simulink model "Template_v5_0_0_2026a_Original"  (R2026a)
settings: Solver=ode4  StopTime=tsim  FixedStep=baseRate  RelTol=1e-6  AbsTol=1e-6
undefined symbols (not defined in the file or in its folder): baseRate, dataRate, DiscIntNeverNeededParam, F_thrusters_BLACK, F_thrusters_BLUE, F_thrusters_RED, home_states_BLACK, home_states_BLUE, home_states_RED, IBLACK, IBLUE, init_states_BLACK, init_states_BLUE, init_states_RED, IRED, K_BLACK, K_BLUE, K_RED, labConsoleIP, mBLACK, mBLUE, mRED, Phase0_End, Phase1_End, Phase2_End, Phase3_End, Phase3_SubPhase1_End, Phase3_SubPhase2_End, Phase3_SubPhase3_End, Phase3_SubPhase4_End, Phase4_End, Phase5_End, platformSelection, PWMFreq, serverRate, simMode, tableDamping_BLACK, tableDamping_BLUE, tableDamping_RED, tableSlope, thrust_decay_BLACK, thrust_decay_BLUE, thrust_decay_RED, thruster_dist2CG_BLACK, thruster_dist2CG_BLUE, thruster_dist2CG_RED, xLength, yLength
libraries: simulink x18, dspinverses x3, nvidiaCommlib x1
(part 6 of 7)

== system Template_v5_0_0_2026a_Original/Simulate Plant Dynamics/RED and ARM Dynamics/RED + ARM/Calculated & Store Measured States/Subsystem3 ==
  dt : Inport
  y : Inport  Port=2
  Constant3 : Constant  Value=0
  Delay1 : Delay  DelayLength=1
  Enabled Subsystem : Subsystem  TreatAsAtomicUnit=on
  Relational Operator : RelationalOperator  Operator=~=  OutDataTypeStr=boolean  RndMeth=Simplest  InputSameDT=off
  Subtract1 : Sum  Inputs=+-
  dy/dt : Outport
  wires:
  Constant3/1 -> Relational Operator/2
  Relational Operator/1 -> Enabled Subsystem/Enable
  Delay1/1 -> Subtract1/2
  dt/1 -> Enabled Subsystem/2(dt)
  Subtract1/1 -> Relational Operator/1
  Enabled Subsystem/1(dy/dt) -> dy/dt/1
  y/1 -> Enabled Subsystem/1(y), Delay1/1, Subtract1/1

== system Template_v5_0_0_2026a_Original/Simulate Plant Dynamics/RED and ARM Dynamics/RED + ARM/Calculated & Store Measured States/Subsystem4 ==
  dt : Inport
  y : Inport  Port=2
  Constant3 : Constant  Value=0
  Delay1 : Delay  DelayLength=1
  Enabled Subsystem : Subsystem  TreatAsAtomicUnit=on
  Relational Operator : RelationalOperator  Operator=~=  OutDataTypeStr=boolean  RndMeth=Simplest  InputSameDT=off
  Subtract1 : Sum  Inputs=+-
  dy/dt : Outport
  wires:
  Constant3/1 -> Relational Operator/2
  Relational Operator/1 -> Enabled Subsystem/Enable
  Delay1/1 -> Subtract1/2
  dt/1 -> Enabled Subsystem/2(dt)
  Subtract1/1 -> Relational Operator/1
  Enabled Subsystem/1(dy/dt) -> dy/dt/1
  y/1 -> Enabled Subsystem/1(y), Delay1/1, Subtract1/1

== system Template_v5_0_0_2026a_Original/Simulate Plant Dynamics/RED and ARM Dynamics/RED + ARM/Calculated & Store Measured States/Subsystem5 ==
  dt : Inport
  y : Inport  Port=2
  Constant3 : Constant  Value=0
  Delay1 : Delay  DelayLength=1
  Enabled Subsystem : Subsystem  TreatAsAtomicUnit=on
  Relational Operator : RelationalOperator  Operator=~=  OutDataTypeStr=boolean  RndMeth=Simplest  InputSameDT=off
  Subtract1 : Sum  Inputs=+-
  dy/dt : Outport
  wires:
  Constant3/1 -> Relational Operator/2
  Relational Operator/1 -> Enabled Subsystem/Enable
  Delay1/1 -> Subtract1/2
  dt/1 -> Enabled Subsystem/2(dt)
  Subtract1/1 -> Relational Operator/1
  Enabled Subsystem/1(dy/dt) -> dy/dt/1
  y/1 -> Enabled Subsystem/1(y), Delay1/1, Subtract1/1

== system Template_v5_0_0_2026a_Original/Simulate Plant Dynamics/RED and ARM Dynamics/RED + ARM/Calculated & Store Measured States/Wrap ==
  Unwrapped Angle : Inport
  Atan2 : Trigonometry  Operator=atan2
  Cos : Trigonometry  Operator=cos
  Sin : Trigonometry
  Wrapped Angle : Outport
  wires:
  Unwrapped Angle/1 -> Sin/1, Cos/1
  Cos/1 -> Atan2/2
  Atan2/1 -> Wrapped Angle/1
  Sin/1 -> Atan2/1

== system Template_v5_0_0_2026a_Original/Simulate Plant Dynamics/RED and ARM Dynamics/RED + ARM/Calculated & Store True States/Wrap ==
  Unwrapped Angle : Inport
  Atan2 : Trigonometry  Operator=atan2
  Cos : Trigonometry  Operator=cos
  Sin : Trigonometry
  Wrapped Angle : Outport
  wires:
  Unwrapped Angle/1 -> Sin/1, Cos/1
  Cos/1 -> Atan2/2
  Atan2/1 -> Wrapped Angle/1
  Sin/1 -> Atan2/1

== system Template_v5_0_0_2026a_Original/Simulate Plant Dynamics/RED and ARM Dynamics/RED + ARM/Data @ Measurement Rate/Calculate True Time Step ==
  Data : Inport
  Time : Inport  Port=2
  Rate : Inport  Port=3
  Constant3 : Constant  Value=0
  Delay1 : Delay  DelayLength=1  InitialCondition=0
  Delay2 : Delay  DelayLength=1  InitialCondition=0
  Demux : Demux  Outputs=[1,5]
  Enabled Subsystem3 : Subsystem  TreatAsAtomicUnit=on
  MATLAB Function : MATLAB Function  TreatAsAtomicUnit=on
  Relational Operator : RelationalOperator  Operator=~=  OutDataTypeStr=boolean  RndMeth=Simplest  InputSameDT=off
  Subtract1 : Sum  Inputs=+-
  Subtract2 : Sum  Inputs=+-
  Terminator : Terminator
  dt_out : Outport
  wires:
  Rate/1 -> MATLAB Function/2(dataRate)
  MATLAB Function/1(dt_out) -> dt_out/1
  Time/1 -> Delay2/1, Subtract1/1
  Enabled Subsystem3/1(dy(t)/dt) -> MATLAB Function/1(dt)
  Data/1 -> Demux/1
  Subtract2/1 -> Relational Operator/1
  Relational Operator/1 -> Enabled Subsystem3/Enable
  Constant3/1 -> Relational Operator/2
  Demux/1 -> Subtract2/1, Delay1/1
  Delay1/1 -> Subtract2/2
  Demux/2 -> Terminator/1
  Subtract1/1 -> Enabled Subsystem3/1(y2-y1)
  Delay2/1 -> Subtract1/2

== system Template_v5_0_0_2026a_Original/Simulate Plant Dynamics/RED and ARM Dynamics/RED + ARM/Data @ Measurement Rate/Enabled Subsystem ==
  In1 : Inport
  Enable : EnablePort
  Out1 : Outport
  wires:
  In1/1 -> Out1/1

== system Template_v5_0_0_2026a_Original/Simulate Plant Dynamics/RED and ARM Dynamics/RED + ARM/Data @ Measurement Rate/Enabled Subsystem1 ==
  ThrustPer_Final : Inport
  Enable : EnablePort
  Out1 : Outport
  wires:
  ThrustPer_Final/1 -> Out1/1

== system Template_v5_0_0_2026a_Original/Simulate Plant Dynamics/RED and ARM Dynamics/RED Only/Calculated & Store Measured States/Subsystem1 ==
  dt : Inport
  y : Inport  Port=2
  Constant3 : Constant  Value=0
  Delay1 : Delay  DelayLength=1
  Enabled Subsystem : Subsystem  TreatAsAtomicUnit=on
  Relational Operator : RelationalOperator  Operator=~=  OutDataTypeStr=boolean  RndMeth=Simplest  InputSameDT=off
  Subtract1 : Sum  Inputs=+-
  dy/dt : Outport
  wires:
  Constant3/1 -> Relational Operator/2
  Relational Operator/1 -> Enabled Subsystem/Enable
  Delay1/1 -> Subtract1/2
  dt/1 -> Enabled Subsystem/2(dt)
  Subtract1/1 -> Relational Operator/1
  Enabled Subsystem/1(dy/dt) -> dy/dt/1
  y/1 -> Enabled Subsystem/1(y), Delay1/1, Subtract1/1

== system Template_v5_0_0_2026a_Original/Simulate Plant Dynamics/RED and ARM Dynamics/RED Only/Calculated & Store Measured States/Subsystem2 ==
  dt : Inport
  y : Inport  Port=2
  Constant3 : Constant  Value=0
  Delay1 : Delay  DelayLength=1
  Enabled Subsystem : Subsystem  TreatAsAtomicUnit=on
  Relational Operator : RelationalOperator  Operator=~=  OutDataTypeStr=boolean  RndMeth=Simplest  InputSameDT=off
  Subtract1 : Sum  Inputs=+-
  dy/dt : Outport
  wires:
  Constant3/1 -> Relational Operator/2
  Relational Operator/1 -> Enabled Subsystem/Enable
  Delay1/1 -> Subtract1/2
  dt/1 -> Enabled Subsystem/2(dt)
  Subtract1/1 -> Relational Operator/1
  Enabled Subsystem/1(dy/dt) -> dy/dt/1
  y/1 -> Delay1/1, Subtract1/1, Enabled Subsystem/1(y)

== system Template_v5_0_0_2026a_Original/Simulate Plant Dynamics/RED and ARM Dynamics/RED Only/Calculated & Store Measured States/Wrap ==
  Unwrapped Angle : Inport
  Atan2 : Trigonometry  Operator=atan2
  Cos : Trigonometry  Operator=cos
  Sin : Trigonometry
  Wrapped Angle : Outport
  wires:
  Unwrapped Angle/1 -> Sin/1, Cos/1
  Cos/1 -> Atan2/2
  Atan2/1 -> Wrapped Angle/1
  Sin/1 -> Atan2/1

== system Template_v5_0_0_2026a_Original/Simulate Plant Dynamics/RED and ARM Dynamics/RED Only/Calculated & Store True States/Wrap ==
  Unwrapped Angle : Inport
  Atan2 : Trigonometry  Operator=atan2
  Cos : Trigonometry  Operator=cos
  Sin : Trigonometry
  Wrapped Angle : Outport
  wires:
  Unwrapped Angle/1 -> Sin/1, Cos/1
  Cos/1 -> Atan2/2
  Atan2/1 -> Wrapped Angle/1
  Sin/1 -> Atan2/1

== system Template_v5_0_0_2026a_Original/Simulate Plant Dynamics/RED and ARM Dynamics/RED Only/Data @ Measurement Rate/Calculate True Time Step ==
  Data : Inport
  Time : Inport  Port=2
  Rate : Inport  Port=3
  Constant3 : Constant  Value=0
  Delay1 : Delay  DelayLength=1  InitialCondition=0
  Delay2 : Delay  DelayLength=1  InitialCondition=0
  Demux : Demux  Outputs=3
  Enabled Subsystem3 : Subsystem  TreatAsAtomicUnit=on
  MATLAB Function : MATLAB Function  TreatAsAtomicUnit=on
  Relational Operator : RelationalOperator  Operator=~=  OutDataTypeStr=boolean  RndMeth=Simplest  InputSameDT=off
  Subtract1 : Sum  Inputs=+-
  Subtract2 : Sum  Inputs=+-
  Terminator : Terminator
  Terminator1 : Terminator
  dt_out : Outport
  wires:
  Demux/3 -> Terminator1/1
  Rate/1 -> MATLAB Function/2(dataRate)
  MATLAB Function/1(dt_out) -> dt_out/1
  Time/1 -> Delay2/1, Subtract1/1
  Enabled Subsystem3/1(dy(t)/dt) -> MATLAB Function/1(dt)
  Data/1 -> Demux/1
  Subtract2/1 -> Relational Operator/1
  Relational Operator/1 -> Enabled Subsystem3/Enable
  Constant3/1 -> Relational Operator/2
  Demux/1 -> Subtract2/1, Delay1/1
  Delay1/1 -> Subtract2/2
  Demux/2 -> Terminator/1
  Subtract1/1 -> Enabled Subsystem3/1(y2-y1)
  Delay2/1 -> Subtract1/2

== system Template_v5_0_0_2026a_Original/Simulate Plant Dynamics/RED and ARM Dynamics/RED Only/Data @ Measurement Rate/Enabled Subsystem ==
  In1 : Inport
  Enable : EnablePort
  Out1 : Outport
  wires:
  In1/1 -> Out1/1

== system Template_v5_0_0_2026a_Original/Simulate Plant Dynamics/RED and ARM Dynamics/RED Only/Data @ Measurement Rate/Enabled Subsystem1 ==
  ThrustPer_Final : Inport
  Enable : EnablePort
  Out1 : Outport
  wires:
  ThrustPer_Final/1 -> Out1/1

== system Template_v5_0_0_2026a_Original/Thruster & Float Control Code/Change BLACK Behavior/Calculate Duty Cycle/Duty Cycle @ PWM/Enabled Subsystem ==
  In1 : Inport
  Enable : EnablePort
  Out1 : Outport
  wires:
  In1/1 -> Out1/1

== system Template_v5_0_0_2026a_Original/Thruster & Float Control Code/Change BLACK Behavior/Calculate Duty Cycle/Duty Cycle @ PWM/Enabled Subsystem1 ==
  ThrustPer_Final : Inport
  Enable : EnablePort
  Out1 : Outport
  wires:
  ThrustPer_Final/1 -> Out1/1

== system Template_v5_0_0_2026a_Original/Thruster & Float Control Code/Change BLUE Behavior/Calculate Duty Cycle/Duty Cycle @ PWM/Enabled Subsystem ==
  In1 : Inport
  Enable : EnablePort
  Out1 : Outport
  wires:
  In1/1 -> Out1/1

== system Template_v5_0_0_2026a_Original/Thruster & Float Control Code/Change BLUE Behavior/Calculate Duty Cycle/Duty Cycle @ PWM/Enabled Subsystem1 ==
  ThrustPer_Final : Inport
  Enable : EnablePort
  Out1 : Outport
  wires:
  ThrustPer_Final/1 -> Out1/1

== system Template_v5_0_0_2026a_Original/Thruster & Float Control Code/Change RED Behavior/Calculate Duty Cycle/Duty Cycle @ PWM/Enabled Subsystem ==
  In1 : Inport
  Enable : EnablePort
  Out1 : Outport
  wires:
  In1/1 -> Out1/1

== system Template_v5_0_0_2026a_Original/Thruster & Float Control Code/Change RED Behavior/Calculate Duty Cycle/Duty Cycle @ PWM/Enabled Subsystem1 ==
  ThrustPer_Final : Inport
  Enable : EnablePort
  Out1 : Outport
  wires:
  ThrustPer_Final/1 -> Out1/1

== system Template_v5_0_0_2026a_Original/1 - Experiment Logic/Phase #3: Experiment/Sub-Phase #1/Desired Position BLACK/Calculate Time since Phase #3 Start/Subsystem ==
  Universal_Time : DataStoreRead  DataStoreName=Univ_Time  IndexOptions=Index vector (dialog)  Indices=1  OutputSizes=1
  Time : Outport  VectorParamsAs1DForOutWhenUnconnected=off
  wires:
  Universal_Time/1 -> Time/1

== system Template_v5_0_0_2026a_Original/1 - Experiment Logic/Phase #3: Experiment/Sub-Phase #1/Desired Position BLUE/Calculate Time since Phase #3 Start/Subsystem ==
  Universal_Time : DataStoreRead  DataStoreName=Univ_Time  IndexOptions=Index vector (dialog)  Indices=1  OutputSizes=1
  Time : Outport  VectorParamsAs1DForOutWhenUnconnected=off
  wires:
  Universal_Time/1 -> Time/1

== system Template_v5_0_0_2026a_Original/1 - Experiment Logic/Phase #3: Experiment/Sub-Phase #1/Desired Position RED/Calculate Time since Phase #3 Start/Subsystem ==
  Universal_Time : DataStoreRead  DataStoreName=Univ_Time  IndexOptions=Index vector (dialog)  Indices=1  OutputSizes=1
  Time : Outport  VectorParamsAs1DForOutWhenUnconnected=off
  wires:
  Universal_Time/1 -> Time/1

== system Template_v5_0_0_2026a_Original/1 - Experiment Logic/Phase #3: Experiment/Sub-Phase #2/Desired Position BLACK/Calculate Time since Phase #3 Start/Subsystem ==
  Universal_Time : DataStoreRead  DataStoreName=Univ_Time  IndexOptions=Index vector (dialog)  Indices=1  OutputSizes=1
  Time : Outport  VectorParamsAs1DForOutWhenUnconnected=off
  wires:
  Universal_Time/1 -> Time/1

== system Template_v5_0_0_2026a_Original/1 - Experiment Logic/Phase #3: Experiment/Sub-Phase #2/Desired Position BLUE/Calculate Time since Phase #3 Start/Subsystem ==
  Universal_Time : DataStoreRead  DataStoreName=Univ_Time  IndexOptions=Index vector (dialog)  Indices=1  OutputSizes=1
  Time : Outport  VectorParamsAs1DForOutWhenUnconnected=off
  wires:
  Universal_Time/1 -> Time/1

== system Template_v5_0_0_2026a_Original/1 - Experiment Logic/Phase #3: Experiment/Sub-Phase #2/Desired Position RED/Calculate Time since Phase #3 Start/Subsystem ==
  Universal_Time : DataStoreRead  DataStoreName=Univ_Time  IndexOptions=Index vector (dialog)  Indices=1  OutputSizes=1
  Time : Outport  VectorParamsAs1DForOutWhenUnconnected=off
  wires:
  Universal_Time/1 -> Time/1

== system Template_v5_0_0_2026a_Original/1 - Experiment Logic/Phase #3: Experiment/Sub-Phase #3/Desired Position BLACK/Calculate Time since Phase #3 Start/Subsystem ==
  Universal_Time : DataStoreRead  DataStoreName=Univ_Time  IndexOptions=Index vector (dialog)  Indices=1  OutputSizes=1
  Time : Outport  VectorParamsAs1DForOutWhenUnconnected=off
  wires:
  Universal_Time/1 -> Time/1

== system Template_v5_0_0_2026a_Original/1 - Experiment Logic/Phase #3: Experiment/Sub-Phase #3/Desired Position BLUE/Calculate Time since Phase #3 Start/Subsystem ==
  Universal_Time : DataStoreRead  DataStoreName=Univ_Time  IndexOptions=Index vector (dialog)  Indices=1  OutputSizes=1
  Time : Outport  VectorParamsAs1DForOutWhenUnconnected=off
  wires:
  Universal_Time/1 -> Time/1

== system Template_v5_0_0_2026a_Original/1 - Experiment Logic/Phase #3: Experiment/Sub-Phase #3/Desired Position RED/Calculate Time since Phase #3 Start/Subsystem ==
  Universal_Time : DataStoreRead  DataStoreName=Univ_Time  IndexOptions=Index vector (dialog)  Indices=1  OutputSizes=1
  Time : Outport  VectorParamsAs1DForOutWhenUnconnected=off
  wires:
  Universal_Time/1 -> Time/1

== system Template_v5_0_0_2026a_Original/1 - Experiment Logic/Phase #3: Experiment/Sub-Phase #4/Desired Position BLACK/Calculate Time since Phase #3 Start/Subsystem ==
  Universal_Time : DataStoreRead  DataStoreName=Univ_Time  IndexOptions=Index vector (dialog)  Indices=1  OutputSizes=1
  Time : Outport  VectorParamsAs1DForOutWhenUnconnected=off
  wires:
  Universal_Time/1 -> Time/1

== system Template_v5_0_0_2026a_Original/1 - Experiment Logic/Phase #3: Experiment/Sub-Phase #4/Desired Position BLUE/Calculate Time since Phase #3 Start/Subsystem ==
  Universal_Time : DataStoreRead  DataStoreName=Univ_Time  IndexOptions=Index vector (dialog)  Indices=1  OutputSizes=1
  Time : Outport  VectorParamsAs1DForOutWhenUnconnected=off
  wires:
  Universal_Time/1 -> Time/1

== system Template_v5_0_0_2026a_Original/1 - Experiment Logic/Phase #3: Experiment/Sub-Phase #4/Desired Position RED/Calculate Time since Phase #3 Start/Subsystem ==
  Universal_Time : DataStoreRead  DataStoreName=Univ_Time  IndexOptions=Index vector (dialog)  Indices=1  OutputSizes=1
  Time : Outport  VectorParamsAs1DForOutWhenUnconnected=off
  wires:
  Universal_Time/1 -> Time/1

== system Template_v5_0_0_2026a_Original/PhaseSpace Camera Code/Use Hardware to Obtain States/Receive and Process Phasespace Data/Experiment Clock/Send Sync. Time/Change BLACK Behavior ==
  Universal Time : Inport
  Action Port : ActionPort  ActionPortLabel=if(u1 == 2 & u2 == 0)
  UDP Send (GUI) : MATLAB Function  TreatAsAtomicUnit=on
  wires:
  Universal Time/1 -> UDP Send (GUI)/1(data)

== system Template_v5_0_0_2026a_Original/PhaseSpace Camera Code/Use Hardware to Obtain States/Receive and Process Phasespace Data/Experiment Clock/Send Sync. Time/Change BLUE Behavior ==
  Universal Time : Inport
  Action Port : ActionPort  ActionPortLabel=if(u1 == 3 & u2 == 0)
  UDP Send (GUI) : MATLAB Function  TreatAsAtomicUnit=on
  wires:
  Universal Time/1 -> UDP Send (GUI)/1(data)

== system Template_v5_0_0_2026a_Original/PhaseSpace Camera Code/Use Hardware to Obtain States/Receive and Process Phasespace Data/Experiment Clock/Send Sync. Time/Change RED Behavior ==
  Universal Time : Inport
  Action Port : ActionPort  ActionPortLabel=if(u1 == 1 & u2 == 0)
  UDP Send (GUI) : MATLAB Function  TreatAsAtomicUnit=on
  wires:
  Universal Time/1 -> UDP Send (GUI)/1(data)

== system Template_v5_0_0_2026a_Original/Simulate Plant Dynamics/RED and ARM Dynamics/RED + ARM/Calculated & Store Measured States/Subsystem3/Enabled Subsystem ==
  y : Inport
  dt : Inport  Port=2
  Enable : EnablePort
  Constant2 : Constant  Value=0.1
  Delay : Delay  DelayLength=1
  MATLAB Function : MATLAB Function  TreatAsAtomicUnit=on
  dy/dt : Outport
  wires:
  Constant2/1 -> MATLAB Function/3(tau)
  dt/1 -> MATLAB Function/2(dt)
  Delay/1 -> MATLAB Function/4(ema_prev)
  MATLAB Function/2(ema) -> Delay/1
  y/1 -> MATLAB Function/1(y)
  MATLAB Function/1(dy) -> dy/dt/1

== system Template_v5_0_0_2026a_Original/Simulate Plant Dynamics/RED and ARM Dynamics/RED + ARM/Calculated & Store Measured States/Subsystem4/Enabled Subsystem ==
  y : Inport
  dt : Inport  Port=2
  Enable : EnablePort
  Constant2 : Constant  Value=0.1
  Delay : Delay  DelayLength=1
  MATLAB Function : MATLAB Function  TreatAsAtomicUnit=on
  dy/dt : Outport
  wires:
  Constant2/1 -> MATLAB Function/3(tau)
  dt/1 -> MATLAB Function/2(dt)
  Delay/1 -> MATLAB Function/4(ema_prev)
  MATLAB Function/2(ema) -> Delay/1
  y/1 -> MATLAB Function/1(y)
  MATLAB Function/1(dy) -> dy/dt/1

== system Template_v5_0_0_2026a_Original/Simulate Plant Dynamics/RED and ARM Dynamics/RED + ARM/Calculated & Store Measured States/Subsystem5/Enabled Subsystem ==
  y : Inport
  dt : Inport  Port=2
  Enable : EnablePort
  Constant2 : Constant  Value=0.1
  Delay : Delay  DelayLength=1
  MATLAB Function : MATLAB Function  TreatAsAtomicUnit=on
  dy/dt : Outport
  wires:
  Constant2/1 -> MATLAB Function/3(tau)
  dt/1 -> MATLAB Function/2(dt)
  Delay/1 -> MATLAB Function/4(ema_prev)
  MATLAB Function/2(ema) -> Delay/1
  y/1 -> MATLAB Function/1(y)
  MATLAB Function/1(dy) -> dy/dt/1

== system Template_v5_0_0_2026a_Original/Simulate Plant Dynamics/RED and ARM Dynamics/RED + ARM/Data @ Measurement Rate/Calculate True Time Step/Enabled Subsystem3 ==
  y2-y1 : Inport
  Enable : EnablePort
  dy(t)/dt : Outport
  wires:
  y2-y1/1 -> dy(t)/dt/1

== system Template_v5_0_0_2026a_Original/Simulate Plant Dynamics/RED and ARM Dynamics/RED Only/Calculated & Store Measured States/Subsystem1/Enabled Subsystem ==
  y : Inport
  dt : Inport  Port=2
  Enable : EnablePort
  Constant2 : Constant  Value=0.1
  Delay : Delay  DelayLength=1
  MATLAB Function : MATLAB Function  TreatAsAtomicUnit=on
  dy/dt : Outport
  wires:
  Constant2/1 -> MATLAB Function/3(tau)
  dt/1 -> MATLAB Function/2(dt)
  Delay/1 -> MATLAB Function/4(ema_prev)
  MATLAB Function/2(ema) -> Delay/1
  y/1 -> MATLAB Function/1(y)
  MATLAB Function/1(dy) -> dy/dt/1

== system Template_v5_0_0_2026a_Original/Simulate Plant Dynamics/RED and ARM Dynamics/RED Only/Calculated & Store Measured States/Subsystem2/Enabled Subsystem ==
  y : Inport
  dt : Inport  Port=2
  Enable : EnablePort
  Constant2 : Constant  Value=0.1
  Delay : Delay  DelayLength=1
  MATLAB Function : MATLAB Function  TreatAsAtomicUnit=on
  dy/dt : Outport
  wires:
  Constant2/1 -> MATLAB Function/3(tau)
  dt/1 -> MATLAB Function/2(dt)
  Delay/1 -> MATLAB Function/4(ema_prev)
  MATLAB Function/2(ema) -> Delay/1
  y/1 -> MATLAB Function/1(y)
  MATLAB Function/1(dy) -> dy/dt/1

== system Template_v5_0_0_2026a_Original/Simulate Plant Dynamics/RED and ARM Dynamics/RED Only/Data @ Measurement Rate/Calculate True Time Step/Enabled Subsystem3 ==
  y2-y1 : Inport
  Enable : EnablePort
  dy(t)/dt : Outport
  wires:
  y2-y1/1 -> dy(t)/dt/1

== matlab function Template_v5_0_0_2026a_Original/Simulate Plant Dynamics/BLACK Dynamics/Calculated & Store Measured States/Subsystem1/Enabled Subsystem/MATLAB Function ==
  data: y input; dy output; dt input; tau input; ema_prev input; ema output
function [dy, ema] = realtime_derivative_ema(y, dt, tau, ema_prev)
    % Compute smoothed derivative using Exponential Moving Average
    %
    % Inputs:
    %   y        : Current measurement
    %   dt       : Time step
    %   tau      : Time constant for EMA filter (larger = more smoothing)
    %   ema_prev : Previous EMA value
    %
    % Outputs:
    %   dy  : Smoothed derivative estimate
    %   ema : Updated EMA value
    
    % Calculate smoothing factor from time constant
    alpha = 1 - exp(-dt ./ tau);
    
    % Update Exponential Moving Average
    ema = alpha .* y + (1 - alpha) .* ema_prev;
    
    % Compute derivative using finite difference on smoothed values
    dy = (ema - ema_prev) ./ dt;
end

== matlab function Template_v5_0_0_2026a_Original/Simulate Plant Dynamics/RED and ARM Dynamics/RED Only/Data @ Measurement Rate/Calculate True Time Step/MATLAB Function ==
  data: dt input; dt_out output; dataRate input
function dt_out = CheckforInvalidTime(dt, dataRate)

    if dt <= 0

        dt_out = dataRate;

    else

        dt_out = dt;

    end


end

== matlab function Template_v5_0_0_2026a_Original/Thruster & Float Control Code/Change BLACK Behavior/Calculate Duty Cycle/MATLAB Function5 ==
  data: H_final output; u_desired input; duty_cycles output; x0 input; thruster_dist2CG_BLACK parameter; F_thrusters_BLACK parameter; max_iters parameter; tol parameter; thrust_decay_BLACK parameter
function [H_final, duty_cycles] = optimize_duty_cycle_with_decay( ...
    u_desired, x0, thruster_dist2CG_BLACK, F_thrusters_BLACK, max_iters, tol, thrust_decay_BLACK)
    %OPTIMIZE_DUTY_CYCLE_WITH_DECAY 
    %   Iteratively optimizes thruster duty cycles while updating thrust decay.
    %
    %   Inputs:
    %       u_desired           - Desired force/torque vector [Fx; Fy; M] (3x1)
    %       x0                  - Initial guess for duty cycles (8x1)
    %       thruster_dist2CG_BLACK- Distances of thrusters from CG (vector, mm)
    %       F_thrusters_BLACK     - Thrust of each thruster (8x1, N): calibrated
    %                             (Calibration tab) or nominal (all eight alike)
    %       max_iters           - Maximum optimization iterations
    %       tol                 - Convergence tolerance (on duty cycles)
    %       thrust_decay_BLACK    - Thrust lost per extra valve open at once: with n
    %                             open, each gives 1 - thrust_decay_BLACK*(n - 1) of
    %                             its thrust alone (thruster calibration, Together)
    %
    %   Outputs:
    %       H_final     - Final H-matrix including thrust decay (3x8)
    %       duty_cycles - Optimized duty cycles (8x1)
    %

    % ---------------------------
    % Initialization
    % ---------------------------
    num_thrusters      = length(x0); %#ok<NASGU> % reserved if needed later
    duty_cycles        = x0;                     % current solution
    thrust_decay_factor = ones(8, 1);            % initial decay (each thruster's share)
    prev_duty_cycles   = duty_cycles + 2*tol;    % force first iteration

    % ---------------------------
    % Iterative optimization
    % ---------------------------
    for iter = 1:max_iters
        % Build system matrix H with current decay factor
        H = MakeHWithDecay(thruster_dist2CG_BLACK, F_thrusters_BLACK, thrust_decay_factor);

        % Solve constrained least squares (box constraints: 0 ≤ x ≤ 1)
        duty_cycles = custom_constrained_least_squares(H, u_desired, duty_cycles);

        % Update each thruster's decay from the current duty cycles
        [thrust_decay_factor, ~] = check_thrust_decay(duty_cycles, thrust_decay_BLACK);

        % Check convergence (∞-norm difference)
        if norm(duty_cycles - prev_duty_cycles, Inf) < tol
            H_final = MakeHWithDecayRecalculateForce(thruster_dist2CG_BLACK, F_thrusters_BLACK, thrust_decay_factor);
            return;
        end

        % Update reference for next iteration
        prev_duty_cycles = duty_cycles;
    end

    % If not converged within max_iters, return final H with last decay
    H_final = MakeHWithDecayRecalculateForce(thruster_dist2CG_BLACK, F_thrusters_BLACK, thrust_decay_factor);
end


% ========================================================================
% Custom Constrained Least Squares Solver
% ========================================================================
function x_opt = custom_constrained_least_squares(H, b, x0)
    %CUSTOM_CONSTRAINED_LEAST_SQUARES
    %   Solves min_x ||H*x - b||^2 subject to 0 <= x <= 1
    %   using projected gradient descent with backtracking line search.
    %
    %   Inputs:
    %       H   - System matrix (3x8)
    %       b   - Desired vector (3x1)
    %       x0  - Initial guess (8x1)
    %
    %   Output:
    %       x_opt - Optimal duty cycle vector (8x1)

    % Parameters
    max_iterations = 100;
    tolerance      = 1e-6;
    alpha          = 0.01;  % initial step size
    beta           = 0.5;   % backtracking factor

    % Initialization
    x      = x0;
    x_prev = x0 + 2*tolerance;

    % Precompute matrices
    HtH = H' * H;
    Htb = H' * b;

    for iter = 1:max_iterations
        % Gradient of ||H*x - b||^2
        gradient = 2 * (HtH*x - Htb);

        % Store objective for comparison
        current_obj = norm(H*x - b)^2;

        % Backtracking line search
        step_size = alpha;
        for ls_iter = 1:20
            x_new = x - step_size * gradient;
            x_new = max(0, min(1, x_new)); % project into [0,1]

            new_obj = norm(H*x_new - b)^2;
            if new_obj < current_obj
                break; % accept step
            else
                step_size = step_size * beta;
            end
        end

        % Update
        x = x_new;

        % Convergence check
        if norm(x - x_prev) < tolerance
            break;
        end

        % Adaptive step size tuning
        if iter > 1 && new_obj < current_obj
            alpha = min(alpha * 1.1, 0.1); % speed up if progress
        else
            alpha = alpha * 0.9;           % slow down otherwise
        end

        % Store for next iteration
        x_prev = x;
    end

    x_opt = x;
end


% ========================================================================
% Construct H-matrix (with decay factor)
% ========================================================================
function H = MakeHWithDecay(thruster_dist2CG, F_thrusters, thrust_decay_factor)
    %MAKEHWITHDECAY
    %   Builds the H matrix that maps thruster duty cycles to [Fx; Fy; M],
    %   applying each thruster's thrust decay (8x1, or one for all).
    %
    %   Outputs H as (3x8)

    % Convert thruster arm distances to meters
    adjusted_dist = thruster_dist2CG / 1000;

    % Thruster directions (X, Y, and moment arm)
    Vec1 = [-1; -1;  0;  0;  1;  1;  0;  0]; % X
    Vec2 = [ 0;  0;  1;  1;  0;  0; -1; -1]; % Y
    Vec3 = adjusted_dist;                    % moment (Z)

    Mat1 = [Vec1, Vec2, Vec3]';

    % Thruster forces (scaled by decay)
    F_decayed = F_thrusters(:) .* thrust_decay_factor(:);

    % Build diagonal scaling
    Mat2 = diag(F_decayed / 2);

    % Final mapping
    H = Mat1 * Mat2;
end


% ========================================================================
% Construct H-matrix (recalculate full force with decay)
% ========================================================================
function H = MakeHWithDecayRecalculateForce(thruster_dist2CG, F_thrusters, thrust_decay_factor)
    %MAKEHWITHDECAYRECALCULATEFORCE
    %   Same as MakeHWithDecay but applies full nominal force scaling.

    adjusted_dist = thruster_dist2CG / 1000;

    Vec1 = [-1; -1;  0;  0;  1;  1;  0;  0];
    Vec2 = [ 0;  0;  1;  1;  0;  0; -1; -1];
    Vec3 = adjusted_dist;

    Mat1 = [Vec1, Vec2, Vec3]';

    F_decayed = F_thrusters(:) .* thrust_decay_factor(:);

    Mat2 = diag(F_decayed);

    H = Mat1 * Mat2;
end


% ========================================================================
% Thrust Decay Update Rule
% ========================================================================
function [thrust_decay_factor, count] = check_thrust_decay(PWMs, decay_per_valve)
    %CHECK_THRUST_DECAY
    %   Each thruster's share of its thrust alone over one PWM period. The
    %   valves share one regulated supply: with n open at once, each gives
    %   max(0, 1 - decay_per_valve*(n - 1)) of its thrust alone (linear, as
    %   the thruster calibration's Together stage measures it). The Teensy
    %   opens every valve at the start of each PWM period and closes each
    %   after its duty cycle, so between two closings the number open is
    %   known, and each thruster's share is the average over its own opening.
    %
    %   Inputs:
    %       PWMs            - Duty cycle vector (8x1)
    %       decay_per_valve - Thrust lost per extra valve open (scalar)
    %
    %   Outputs:
    %       thrust_decay_factor - Each thruster's share of its thrust (8x1)
    %       count               - Number of active thrusters

    % Normalize if needed
    if max(PWMs) > 1
        PWMs = PWMs / max(PWMs);
    end
    duty = max(PWMs(:), 0);

    % Active thrusters
    count = sum(duty > 0);

    % The instants the valves close, in order
    closing = sort(duty);

    thrust_decay_factor = ones(8, 1);
    for i = 1:8
        if duty(i) > 0
            share = 0;
            t0 = 0;
            for k = 1:8
                t1 = min(closing(k), duty(i));
                if t1 > t0
                    n_open = sum(duty >= t1);   % valves open from t0 to t1
                    share = share + (t1 - t0) * max(0, 1 - decay_per_valve*(n_open - 1));
                    t0 = t1;
                end
            end
            thrust_decay_factor(i) = share / duty(i);
        end
    end
end

== matlab function Template_v5_0_0_2026a_Original/Simulate Plant Dynamics/RED and ARM Dynamics/RED + ARM/Calculated & Store Measured States/Subsystem4/Enabled Subsystem/MATLAB Function ==
  data: y input; dy output; dt input; tau input; ema_prev input; ema output
function [dy, ema] = realtime_derivative_ema(y, dt, tau, ema_prev)
    % Compute smoothed derivative using Exponential Moving Average
    %
    % Inputs:
    %   y        : Current measurement
    %   dt       : Time step
    %   tau      : Time constant for EMA filter (larger = more smoothing)
    %   ema_prev : Previous EMA value
    %
    % Outputs:
    %   dy  : Smoothed derivative estimate
    %   ema : Updated EMA value
    
    % Calculate smoothing factor from time constant
    alpha = 1 - exp(-dt ./ tau);
    
    % Update Exponential Moving Average
    ema = alpha .* y + (1 - alpha) .* ema_prev;
    
    % Compute derivative using finite difference on smoothed values
    dy = (ema - ema_prev) ./ dt;
end

== matlab function Template_v5_0_0_2026a_Original/PhaseSpace Camera Code/Use Hardware to Obtain States/Store RED Data/Subsystem1/Enabled Subsystem/MATLAB Function ==
  data: y input; dy output; dt input; tau input; ema_prev input; ema output
function [dy, ema] = realtime_derivative_ema(y, dt, tau, ema_prev)
    % Compute smoothed derivative using Exponential Moving Average
    %
    % Inputs:
    %   y        : Current measurement
    %   dt       : Time step
    %   tau      : Time constant for EMA filter (larger = more smoothing)
    %   ema_prev : Previous EMA value
    %
    % Outputs:
    %   dy  : Smoothed derivative estimate
    %   ema : Updated EMA value
    
    % Calculate smoothing factor from time constant
    alpha = 1 - exp(-dt ./ tau);
    
    % Update Exponential Moving Average
    ema = alpha .* y + (1 - alpha) .* ema_prev;
    
    % Compute derivative using finite difference on smoothed values
    dy = (ema - ema_prev) ./ dt;
end

== matlab function Template_v5_0_0_2026a_Original/Simulate Plant Dynamics/RED and ARM Dynamics/RED Only/Calculated & Store Measured States/Subsystem1/Enabled Subsystem/MATLAB Function ==
  data: y input; dy output; dt input; tau input; ema_prev input; ema output
function [dy, ema] = realtime_derivative_ema(y, dt, tau, ema_prev)
    % Compute smoothed derivative using Exponential Moving Average
    %
    % Inputs:
    %   y        : Current measurement
    %   dt       : Time step
    %   tau      : Time constant for EMA filter (larger = more smoothing)
    %   ema_prev : Previous EMA value
    %
    % Outputs:
    %   dy  : Smoothed derivative estimate
    %   ema : Updated EMA value
    
    % Calculate smoothing factor from time constant
    alpha = 1 - exp(-dt ./ tau);
    
    % Update Exponential Moving Average
    ema = alpha .* y + (1 - alpha) .* ema_prev;
    
    % Compute derivative using finite difference on smoothed values
    dy = (ema - ema_prev) ./ dt;
end

== matlab function Template_v5_0_0_2026a_Original/Simulate Plant Dynamics/BLACK Dynamics/Calculated & Store Measured States/Subsystem2/Enabled Subsystem/MATLAB Function ==
  data: y input; dy output; dt input; tau input; ema_prev input; ema output
function [dy, ema] = realtime_derivative_ema(y, dt, tau, ema_prev)
    % Compute smoothed derivative using Exponential Moving Average
    %
    % Inputs:
    %   y        : Current measurement
    %   dt       : Time step
    %   tau      : Time constant for EMA filter (larger = more smoothing)
    %   ema_prev : Previous EMA value
    %
    % Outputs:
    %   dy  : Smoothed derivative estimate
    %   ema : Updated EMA value
    
    % Calculate smoothing factor from time constant
    alpha = 1 - exp(-dt ./ tau);
    
    % Update Exponential Moving Average
    ema = alpha .* y + (1 - alpha) .* ema_prev;
    
    % Compute derivative using finite difference on smoothed values
    dy = (ema - ema_prev) ./ dt;
end

== matlab function Template_v5_0_0_2026a_Original/Live Data Streams/Live Stream 1/Stream ==
  data: u input; t input; whoAmI input; isSim input; streamLabel parameter; labConsoleIP parameter
function streamData(u, t, whoAmI, isSim, streamLabel, labConsoleIP)
%STREAMDATA Sends this block's input to the SPOT Console's live plot, every step.
%   Its name in the plot is the name of what is connected (e.g. a Data Store Read's data store)
%   or the name typed into the block (double-click it). See help spot.hardware.liveStream.
%#codegen
spot.hardware.liveStream(streamLabel, t, u, whoAmI, isSim, labConsoleIP);
end

== matlab function Template_v5_0_0_2026a_Original/Simulate Plant Dynamics/BLACK Dynamics/Data @ Measurement Rate/Calculate True Time Step/MATLAB Function ==
  data: dt input; dt_out output; dataRate input
function dt_out = CheckforInvalidTime(dt, dataRate)

    if dt <= 0

        dt_out = dataRate;

    else

        dt_out = dt;

    end


end

== matlab function Template_v5_0_0_2026a_Original/4 - Control/Custom Control (ARM)/Calculate PWM ==
  data: u input; y output
function y = PlaceholderControl(u)

    y = u;

end

== matlab function Template_v5_0_0_2026a_Original/Simulate Plant Dynamics/BLUE Dynamics/Calculated & Store Measured States/Subsystem1/Enabled Subsystem/MATLAB Function ==
  data: y input; dy output; dt input; tau input; ema_prev input; ema output
function [dy, ema] = realtime_derivative_ema(y, dt, tau, ema_prev)
    % Compute smoothed derivative using Exponential Moving Average
    %
    % Inputs:
    %   y        : Current measurement
    %   dt       : Time step
    %   tau      : Time constant for EMA filter (larger = more smoothing)
    %   ema_prev : Previous EMA value
    %
    % Outputs:
    %   dy  : Smoothed derivative estimate
    %   ema : Updated EMA value
    
    % Calculate smoothing factor from time constant
    alpha = 1 - exp(-dt ./ tau);
    
    % Update Exponential Moving Average
    ema = alpha .* y + (1 - alpha) .* ema_prev;
    
    % Compute derivative using finite difference on smoothed values
    dy = (ema - ema_prev) ./ dt;
end

== matlab function Template_v5_0_0_2026a_Original/Simulate Plant Dynamics/BLACK Dynamics/Dynamics Model for BLACK/MATLAB Function ==
  data: control_inputs input; position input; velocity input; floating input; x_ddot output; mBLACK parameter; IBLACK parameter; tableSlope parameter; tableDamping_BLACK parameter
function x_ddot = BLACK_dynamics(control_inputs, position, velocity, floating, mBLACK, IBLACK, tableSlope, tableDamping_BLACK)

%#codegen
% Fully define the size of x_ddot() for code generation:
x_ddot     = zeros(3,1);

% Extract the control inputs from the control_input vector:
Fx        = control_inputs(1);              % [N]
Fy        = control_inputs(2);              % [N]
Tz        = control_inputs(3);              % [N.m]

% Calculate the state acceleration vector:
x_ddot(1) = Fx/mBLACK;                      % [m/s^2]
x_ddot(2) = Fy/mBLACK;                      % [m/s^2]
x_ddot(3) = Tz/IBLACK;                      % [rad/s^2]
% The table's pull (the Calibration tab; spot.dynamics.tableSlope): while the platform floats
% (FLOATING: Float_State), it slides down the table's slope and its air bearings drag it. POSITION
% and VELOCITY are the previous step's (Previous Position, Previous Velocity). tableSlope is all
% zeros on a level table (Scenario: Table Slope off, or no calibration).
if floating ~= 0
    x_ddot(1:2) = x_ddot(1:2) + spot.dynamics.tableSlope(position, velocity, tableSlope, tableDamping_BLACK);
end


end

== matlab function Template_v5_0_0_2026a_Original/Simulate Plant Dynamics/BLUE Dynamics/BLUE  Dynamics Model/MATLAB Function ==
  data: control_inputs input; position input; velocity input; floating input; x_ddot output; mBLUE parameter; IBLUE parameter; tableSlope parameter; tableDamping_BLUE parameter
function x_ddot = BLUE_dynamics(control_inputs, position, velocity, floating, mBLUE, IBLUE, tableSlope, tableDamping_BLUE)%#codegen
% Fully define the size of x_ddot() for code generation:
x_ddot     = zeros(3,1);

% Extract the control inputs from the control_input vector:
Fx        = control_inputs(1);              % [N]
Fy        = control_inputs(2);              % [N]
Tz        = control_inputs(3);              % [N.m]

% Calculate the state acceleration vector:
x_ddot(1) = Fx/mBLUE;                      % [m/s^2]
x_ddot(2) = Fy/mBLUE;                      % [m/s^2]
x_ddot(3) = Tz/IBLUE;                      % [rad/s^2]
% The table's pull (the Calibration tab; spot.dynamics.tableSlope): while the platform floats
% (FLOATING: Float_State), it slides down the table's slope and its air bearings drag it. POSITION
% and VELOCITY are the previous step's (Previous Position, Previous Velocity). tableSlope is all
% zeros on a level table (Scenario: Table Slope off, or no calibration).
if floating ~= 0
    x_ddot(1:2) = x_ddot(1:2) + spot.dynamics.tableSlope(position, velocity, tableSlope, tableDamping_BLUE);
end


end

== matlab function Template_v5_0_0_2026a_Original/Thruster & Float Control Code/MATLAB Function2 ==
  data: duty_cycles input; packet output; air_bearing input
function packet = pack_command(duty_cycles, air_bearing)

    %#codegen
    %
    % Inputs:
    %   duty_cycles : 8x1 single, 0-100
    %   air_bearing : scalar single, 0 or 1
    %
    % Output:
    %   packet : 37x1 uint8
    %

    packet = zeros(37, 1, 'uint8');

    % =====================================================
    % Sync byte
    % =====================================================
    packet(1) = uint8(170);   % 0xAA

    % =====================================================
    % Eight thruster duties
    % Bytes 2-33
    % =====================================================
    for i = 1:8

        dbytes = typecast(single(duty_cycles(i)), 'uint8');

        base = uint32(2 + (i-1)*4);

        packet(base    ) = dbytes(1);
        packet(base + 1) = dbytes(2);
        packet(base + 2) = dbytes(3);
        packet(base + 3) = dbytes(4);

    end

    % =====================================================
    % Air bearing / puck
    % Bytes 34-37
    % =====================================================
    abytes = typecast(single(air_bearing), 'uint8');

    packet(34) = abytes(1);
    packet(35) = abytes(2);
    packet(36) = abytes(3);
    packet(37) = abytes(4);

end

== matlab function Template_v5_0_0_2026a_Original/Simulate Plant Dynamics/BLUE Dynamics/Calculated & Store Measured States/Subsystem2/Enabled Subsystem/MATLAB Function ==
  data: y input; dy output; dt input; tau input; ema_prev input; ema output
function [dy, ema] = realtime_derivative_ema(y, dt, tau, ema_prev)
    % Compute smoothed derivative using Exponential Moving Average
    %
    % Inputs:
    %   y        : Current measurement
    %   dt       : Time step
    %   tau      : Time constant for EMA filter (larger = more smoothing)
    %   ema_prev : Previous EMA value
    %
    % Outputs:
    %   dy  : Smoothed derivative estimate
    %   ema : Updated EMA value
    
    % Calculate smoothing factor from time constant
    alpha = 1 - exp(-dt ./ tau);
    
    % Update Exponential Moving Average
    ema = alpha .* y + (1 - alpha) .* ema_prev;
    
    % Compute derivative using finite difference on smoothed values
    dy = (ema - ema_prev) ./ dt;
end

== matlab function Template_v5_0_0_2026a_Original/Simulate Plant Dynamics/BLUE Dynamics/Data @ Measurement Rate/Calculate True Time Step/MATLAB Function ==
  data: dt input; dt_out output; dataRate input
function dt_out = CheckforInvalidTime(dt, dataRate)

    if dt <= 0

        dt_out = dataRate;

    else

        dt_out = dt;

    end


end
